simulink model "EV6_LUT_FourWheel_EV6Battery77p4kWh_PowerCorrected"  (R2024a)
settings: Solver=ode4  StartTime=0  StopTime=60  FixedStep=0.001  RelTol=1e-3
PreLoadFcn:
  | VSS_BICYCLE=Simulink.Variant('Dual=0');
  | VSS_DUAL=Simulink.Variant('Dual=1');
  | Dual=1;
  | load('DriveCycle2.mat')
PostLoadFcn:
  | if any(exist('dsrtsu_mdlpostloadfcn', 'file') ~= 0), dsrtsu_mdlpostloadfcn('Execute', bdroot); end
InitFcn:
  | , if any(exist('rtifpga_mdlclblib', 'file') ~= 0), rtifpga_mdlclblib('Init', bdroot); end,
  | , if any(exist('dsmpb_private', 'file') ~= 0), dsmpb_private('dsmpb_mdlclblib', 'Init', bdroot); end,
  | load('DriveCycle2.mat')
model workspace (MAT data in the model file):
  DiffRatio = 10.65
  EV6_2023_BattBranchCapacity_Ah = 55.5236728838
  EV6_2023_BattEnergy_kWh = 77.4
  EV6_2023_BattNominalVoltage_V = 697
  EV6_2023_BattNumCellsParallel = 2
  EV6_2023_BattNumCellsSeries = 192
  EV6_2023_BattOpenVoltCapBpts = [0 0.1 0.2 0.3 0.4 0.5 0.6 0.7 0.8 0.9 1]
  EV6_2023_BattOpenVoltTbl = [2.96762142548 3.40364281191 3.47417488548 3.54470541822 3.61523441014 3.68576186124 3.75628777151 3.82681214095 3.94527005036 4.07101207308 4.2120755254]
  EV6_2023_BattPackCapacity_Ah = 111.047345768
  EV6_2023_BattResistSocBpts = [0 0.2 0.4 0.6 0.8 1]
  EV6_2023_BattResistTbl = [0.0163620057716 0.0118174152018 0.00807187352333 0.00375663957972 0.00266904525531 0.00103635901355 0.0019014404175 0.0172368903217 0.0121226074867 0.00758541551769 0.00474065349228 0.00337561163613 ... (42 elements, 7x6)]
  EV6_2023_BattResistTempBpts = [243.1 253.1 263.1 273.1 283.1 298.1 313.1]
  EV6_2023_InitialPackOCV_V = 726.471714233
  EV6_2023_InitialSOC = 0.638878863672
  EV6_BattCellCapacity_Ah = 60.3
  EV6_BattInitialSOC = 0.638878863672
  EV6_BattOCV_Cell_V = [2.96762142548 3.40364281191 3.47417488548 3.54470541822 3.61523441014 3.68576186124 3.75628777151 3.82681214095 3.94527005036 4.07101207308 4.2120755254]
  EV6_BattOCV_SOC = [0 0.1 0.2 0.3 0.4 0.5 0.6 0.7 0.8 0.9 1]
  EV6_BattPackCapacity_Ah = 120.6
  EV6_BattParallelCells = 2
  EV6_BattResistanceSOC = [0 0.2 0.4 0.6 0.8 1]
  EV6_BattResistanceTable_Ohm = [0.0163620057716 0.0118174152018 0.00807187352333 0.00375663957972 0.00266904525531 0.00103635901355 0.0019014404175 0.0172368903217 0.0121226074867 0.00758541551769 0.00474065349228 0.00337561163613 ... (42 elements, 7x6)]
  EV6_BattResistanceTemp_K = [243.1 253.1 263.1 273.1 283.1 298.1 313.1]
  EV6_BattSeriesCells = 192
  EV6_FinalDriveRatio = 10.65
  EV6_TargetPackResistance_Ohm = 0.132763804608
  Gas = 0.383333333333
undefined symbols (not defined in the file): accel_bp_mps2, AccelCmd, ActTqLF_Nm_, ActTqLR_Nm_, ActTqRF_Nm_, ActTqRR_Nm_, BattChargeLimitMaxPwr, BattChargeLimitSocBpts, BattChargeLimitTbl, BattDischargeLimitSocBpts, BattDischargeLimitTbl, BattDischargeMaxPwr, BrakeMaxPrs, BrakeMaxTrq, ChassisDistCg2FrontAxle, ChassisDistCg2RearAxle, ChassisVehMass, CltchCmd, CoastDown, DecelCmd, DiscIntNeverNeededParam, EnvGravCnst, EnvPrs, EnvTemp, EV6_RegenTorqueGain, EV6_TractionTorqueGain, front_share_regen_3d, front_share_traction_3d, FuelSpecificGrav, GearCmd, h, InitStates, lgSw, limitedMCT, MCT, MtrEffSpdBpts, MtrEffTbl, MtrEffTrqBpts, MtrPwrMax, MtrTrqMax, out_1, pMCT, RealSimPara, Ref_speed, Ref_time, regen_torque_bp_Nm, speed_bp_kph, SteeringCmd, SupvsryCtrlRegenBrkCutOffTbl, SupvsryCtrlRegenSpdBpts, TestScnrioCycleNum, traction_torque_bp_Nm, US06, VEH
libraries: VSIGenLib x65, simulink x54, etargetslib x38, dsmpblib x24, vehdynlibtire x12, autolibshared x11, vehdynlibsuspension x7, vehdynlibtirecommon x7, autolibpowerinfoutils x6, autolibutils x5, autolibsharedcoupling x4, autolibmappedmotor x4
(part 11 of 19)

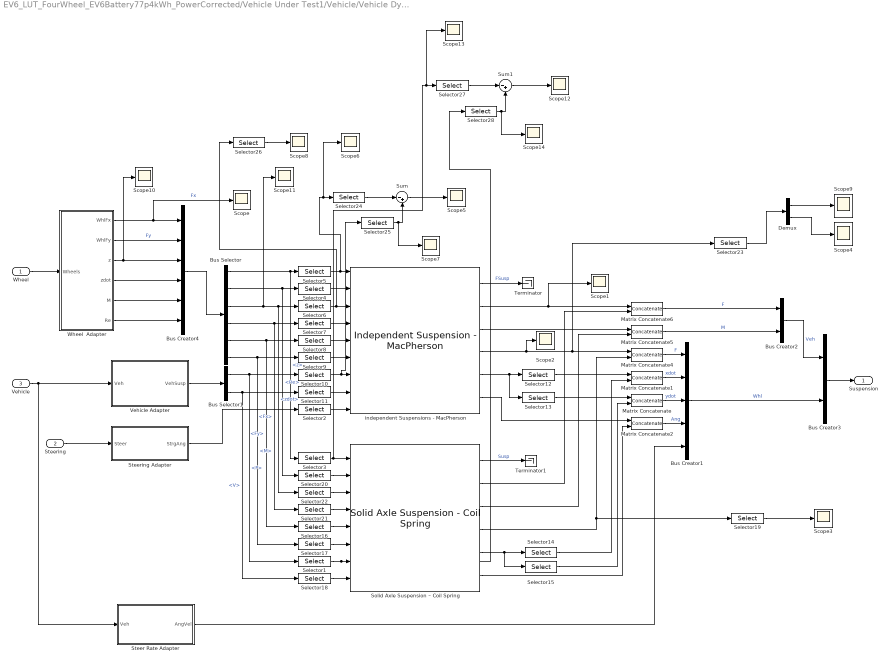
== system EV6_LUT_FourWheel_EV6Battery77p4kWh_PowerCorrected/Vehicle Under Test1/Vehicle/Vehicle Dynamics/Vehicle 14DOF/Suspension/MacPherson Front Suspension Solid Axle Rear Suspension ==
  Wheel : Inport
  Steering : Inport  Port=2
  Vehicle : Inport  Port=3
  Bus Creator1 : BusCreator  Inputs=5
  Bus Creator2 : BusCreator  Inputs=2
  Bus Creator3 : BusCreator  Inputs=2
  Bus Creator4 : BusCreator  Inputs=6
  Bus Selector : BusSelector  OutputSignals=z,Re,zdot,Fx,Fy,M
  Bus Selector1 : BusSelector  OutputSignals=P,V
  Demux : Demux  Outputs=2
  Matrix Concatenate{,1..2,4..6} (6 alike) : Concatenate  Mode=Multidimensional array  ConcatenateDimension=2
  Scope{,1..14} (15 alike) : Scope
  Selector1 : Selector  NumberOfDimensions=2  IndexOptions=Select all,Index vector (dialog)  Indices=[1 2],[3 4]  OutputSizes=1,1
  Selector10 : Selector  NumberOfDimensions=2  IndexOptions=Select all,Index vector (dialog)  Indices=[1 2],[1 2]  OutputSizes=1,1
  Selector11 : Selector  NumberOfDimensions=2  IndexOptions=Select all,Index vector (dialog)  Indices=[1 2],[1 2]  OutputSizes=1,1
  Selector12 : Selector  NumberOfDimensions=2  InputPortWidth=3  IndexOptions=Index vector (dialog),Select all  Indices=1,1  OutputSizes=1,1
  Selector13 : Selector  NumberOfDimensions=2  InputPortWidth=3  IndexOptions=Index vector (dialog),Select all  Indices=2,1  OutputSizes=1,1
  Selector14 : Selector  NumberOfDimensions=2  InputPortWidth=3  IndexOptions=Index vector (dialog),Select all  Indices=1,1  OutputSizes=1,1
  Selector15 : Selector  NumberOfDimensions=2  InputPortWidth=3  IndexOptions=Index vector (dialog),Select all  Indices=2,1  OutputSizes=1,1
  Selector{3,16,20..22} (5 alike) : Selector  IndexOptions=Index vector (dialog)  Indices=[3 4]  OutputSizes=1
  Selector17 : Selector  NumberOfDimensions=2  IndexOptions=Select all,Index vector (dialog)  Indices=[1 2],[3 4]  OutputSizes=1,1
  Selector18 : Selector  NumberOfDimensions=2  IndexOptions=Select all,Index vector (dialog)  Indices=[1 2],[3 4]  OutputSizes=1,1
  Selector19 : Selector  NumberOfDimensions=2  InputPortWidth=3  IndexOptions=Index vector (dialog),Select all  Indices=3,1  OutputSizes=1,1
  Selector{2,4..8} (6 alike) : Selector  IndexOptions=Index vector (dialog)  Indices=[1 2]  OutputSizes=1
  Selector23 : Selector  NumberOfDimensions=2  InputPortWidth=3  IndexOptions=Index vector (dialog),Select all  Indices=3,1  OutputSizes=1,1
  Selector24 : Selector  IndexOptions=Index vector (dialog)  Indices=[1]  OutputSizes=1
  Selector25 : Selector  NumberOfDimensions=2  IndexOptions=Index vector (dialog),Index vector (dialog)  Indices=[3],[1]  OutputSizes=1,1
  Selector26 : Selector  IndexOptions=Index vector (dialog)  Indices=[1]  OutputSizes=1
  Selector27 : Selector  IndexOptions=Index vector (dialog)  Indices=[1]  OutputSizes=1
  Selector28 : Selector  NumberOfDimensions=2  IndexOptions=Index vector (dialog),Index vector (dialog)  Indices=[3],[1]  OutputSizes=1,1
  Selector9 : Selector  NumberOfDimensions=2  IndexOptions=Select all,Index vector (dialog)  Indices=[1 2],[1 2]  OutputSizes=1,1
  Solid Axle Suspension – Coil Spring : vehdynlibsuspension/Solid Axle Suspension - Coil Spring  NumAxl=1  NumWhlsByAxl=2  StrgEnByAxl=0  WhlNumVec="[1  2]"  AxleNumVec="[1  1]"  SuspTypesByAxle=[1]  SuspImage=suspsacoil.png  AxlIxx=62  AxlM=160  TrackCoords=[0 0;1.9*[-1 1]/2;0 0]  SuspCoords=[0 0;1.9*[-1 1]/2;0 0]  KzWhlAxl=138031  F0zWhlAxl=5003*1  CzWhlAxl=11490  IdealSuspEn=on  IdealSuspAxles=[1]  Kz=52451*1  F0z=5003*1  Cz=5565*1  Hmax=0.32  Toe=0.  RollStrgSlp=0.  ToeStrgSlp=0  Caster=0.  CasterHslp=0.  CasterStrgSlp=0.01  Camber=0.  CamberHslp=0.  CamberStrgSlp=0.01  StrgHgtSlp=0.1432  MappedSuspEn=off  MappedSuspAxles="[1  2]"  f_susp_axl_bp=[1 2]  f_susp_dz_bp=[-0.15 -0.14 -0.13 -0.12 -0.11 -0.10 -0.09 -0.08 -0.07 -0.06 -0.05 -0.04 -0.03 -0.02 -0.01 0.00 0.01 0.02 0.03 0.04 0.05 0.06 0.07 0.08 0.09 0.10 0.11 0.12 0.13 0.14 0.15]  f_susp_dzdot_bp=[-0.15 -0.14 -0.13 -0.12 -0.11 -0.10 -0.09 -0.08 -0.07 -0.06 -0.05 -0.04 -0.03 -0.02 -0.01 0.00 0.01 0.02 0.03 0.04 0.05 0.06 0.07 0.08 0.09 0.10 0.11 0.12 0.13 0.14 0.15]  f_susp_fmz=zeros(31,31,61,2,4)  f_susp_geom=zeros(31,61,2,3)  f_susp_strgdelta_bp=[-30,-29,-28,-27,-26,-25,-24,-23,-22,-21,-20,-19,-18,-17,-16,-15,-14,-13,-12,-11,-10,-9,-8,-7,-6,-5,-4,-3,-2,-1,0,1,2,3,4,5,6,7,8,9,10,11,12,13,14,15,16,17,18,19,20,21,22,23,24,25,26,27,28,29,30]
  Steer Rate Adapter : Subsystem
  Steering Adapter : Subsystem
  Sum : Sum  Inputs=|-+
  Sum1 : Sum  Inputs=|-+
  Terminator : Terminator
  Terminator1 : Terminator
  Vehicle Adapter : Subsystem
  Wheel  Adapter : Subsystem
  independent Suspensions - MacPherson : vehdynlibsuspension/Independent Suspension - MacPherson  ActiveDampEn=off  NumAxl=1  NumWhlsByAxl=2  StrgEnByAxl=1  AntiSwayEnByAxl=1  WhlNumVec="[1  2]"  AxleNumVec="[1  1]"  SuspTypesByAxle=[1]  SuspImage=suspmacp.png  IdealSuspEn=on  IdealSuspAxles=[1]  Kz=52451*1  F0z=5003*1  Cz=5565*1  Hmax=0.32  f_act_susp_cz=[10000 10000;10000 10000]  f_act_susp_duty_bpt=[0 1]  f_act_susp_zdot_bpt=[-1 1]  Toe=0.  RollStrgSlp=0.  ToeStrgSlp=0.  Caster=0.  CasterHslp=0.  CasterStrgSlp=0.  Camber=0.  CamberHslp=0.  CamberStrgSlp=0.  StrgHgtSlp=0.1432  MappedSuspEn=off  MappedSuspAxles="[1  2]"  f_susp_axl_bp=[1 2]  f_susp_dz_bp=[-0.15 -0.14 -0.13 -0.12 -0.11 -0.10 -0.09 -0.08 -0.07 -0.06 -0.05 -0.04 -0.03 -0.02 -0.01 0.00 0.01 0.02 0.03 0.04 0.05 0.06 0.07 0.08 0.09 0.10 0.11 0.12 0.13 0.14 0.15]  f_susp_dzdot_bp=[-0.15 -0.14 -0.13 -0.12 -0.11 -0.10 -0.09 -0.08 -0.07 -0.06 -0.05 -0.04 -0.03 -0.02 -0.01 0.00 0.01 0.02 0.03 0.04 0.05 0.06 0.07 0.08 0.09 0.10 0.11 0.12 0.13 0.14 0.15]  f_susp_fmz=zeros(31,31,61,2,4)  f_susp_geom=zeros(31,61,2,3)  f_susp_strgdelta_bp=[-30,-29,-28,-27,-26,-25,-24,-23,-22,-21,-20,-19,-18,-17,-16,-15,-14,-13,-12,-11,-10,-9,-8,-7,-6,-5,-4,-3,-2,-1,0,1,2,3,4,5,6,7,8,9,10,11,12,13,14,15,16,17,18,19,20,21,22,23,24,25,26,27,28,29,30]  AntiSwayR=0.2  AntiSwayNtrlAng=0.5236  AntiSwayTrsK=8e+02
  Suspension : Outport  VectorParamsAs1DForOutWhenUnconnected=off
  wires:
  Steer Rate Adapter/1(AngVel) -> Bus Creator1/5
  Solid Axle Suspension – Coil Spring/5 -> Selector14/1, Selector15/1
  Solid Axle Suspension – Coil Spring/1 -> Terminator1/1  "Susp"
  Bus Selector/3 -> Scope11/1, Selector6/1, Selector22/1  "<zdot>"
  Selector22/1 -> Solid Axle Suspension – Coil Spring/3
  Vehicle/1 -> Vehicle Adapter/1(Veh), Steer Rate Adapter/1(Veh)
  Solid Axle Suspension – Coil Spring/3 -> Matrix Concatenate5/2
  Selector21/1 -> Solid Axle Suspension – Coil Spring/4
  Wheel  Adapter/6(Re) -> Bus Creator4/6
  Selector20/1 -> Solid Axle Suspension – Coil Spring/2
  Selector18/1 -> Solid Axle Suspension – Coil Spring/8
  Selector17/1 -> Solid Axle Suspension – Coil Spring/6
  Selector16/1 -> Solid Axle Suspension – Coil Spring/5
  Solid Axle Suspension – Coil Spring/2 -> Matrix Concatenate6/2
  Matrix Concatenate6/1 -> Bus Creator2/1  "F"
  Matrix Concatenate5/1 -> Bus Creator2/2  "M"
  Solid Axle Suspension – Coil Spring/4 -> Selector19/1, Matrix Concatenate4/2
  Matrix Concatenate4/1 -> Bus Creator1/1  "F"
  Solid Axle Suspension – Coil Spring/6 -> Matrix Concatenate2/2
  Matrix Concatenate2/1 -> Bus Creator1/4  "Ang"
  Selector14/1 -> Matrix Concatenate1/2
  Matrix Concatenate1/1 -> Bus Creator1/2  "xdot"
  Selector15/1 -> Matrix Concatenate/2
  Selector13/1 -> Matrix Concatenate/1
  Selector11/1 -> independent Suspensions - MacPherson/8
  Selector10/1 -> Selector25/1, independent Suspensions - MacPherson/7
  Selector9/1 -> independent Suspensions - MacPherson/6
  Selector8/1 -> independent Suspensions - MacPherson/5
  Selector7/1 -> independent Suspensions - MacPherson/4
  Selector6/1 -> Selector26/1, independent Suspensions - MacPherson/3
  Selector5/1 -> Scope6/1, Selector24/1, independent Suspensions - MacPherson/1
  Selector4/1 -> independent Suspensions - MacPherson/2
  Selector2/1 -> independent Suspensions - MacPherson/9
  Bus Selector/2 -> Selector4/1, Selector20/1  "<Re>"
  Wheel  Adapter/5(M) -> Bus Creator4/5
  Wheel  Adapter/4(zdot) -> Bus Creator4/4
  Wheel  Adapter/3(z) -> Scope10/1, Bus Creator4/3
  Wheel/1 -> Wheel  Adapter/1(Wheels)
  Wheel  Adapter/1(WhlFx) -> Bus Creator4/1, Scope/1  "Fx"
  Wheel  Adapter/2(WhlFy) -> Bus Creator4/2  "Fy"
  Bus Creator4/1 -> Bus Selector/1
  Steering Adapter/1(StrgAng) -> Selector2/1
  Bus Creator2/1 -> Bus Creator3/1  "Veh"
  independent Suspensions - MacPherson/3 -> Matrix Concatenate5/1
  independent Suspensions - MacPherson/2 -> Matrix Concatenate6/1, Scope1/1
  Vehicle Adapter/1(VehSusp) -> Bus Selector1/1
  Bus Selector/4 -> Selector21/1, Selector7/1  "<Fx>"
  independent Suspensions - MacPherson/1 -> Terminator/1  "FSusp"
  independent Suspensions - MacPherson/4 -> Selector23/1, Matrix Concatenate4/1, Scope2/1
  Selector12/1 -> Matrix Concatenate1/1
  independent Suspensions - MacPherson/6 -> Matrix Concatenate2/1
  independent Suspensions - MacPherson/5 -> Selector13/1, Selector12/1
  Matrix Concatenate/1 -> Bus Creator1/3  "ydot"
  Bus Selector1/1 -> Selector1/1, Selector10/1  "<P>"
  Steering/1 -> Steering Adapter/1(Steer)
  Bus Selector/1 -> Selector5/1, Selector3/1  "<z>"
  Bus Selector/5 -> Selector16/1, Selector8/1  "<Fy>"
  Bus Selector/6 -> Selector17/1, Selector9/1  "<M>"
  Bus Selector1/2 -> Selector18/1, Selector11/1  "<V>"
  Bus Creator1/1 -> Bus Creator3/2  "Whl"
  Bus Creator3/1 -> Suspension/1
  Selector19/1 -> Scope3/1
  Selector23/1 -> Demux/1
  Selector24/1 -> Sum/1
  Selector25/1 -> Scope7/1, Sum/2
  Sum/1 -> Scope5/1
  Selector26/1 -> Scope8/1
  Demux/1 -> Scope9/1
  Demux/2 -> Scope4/1
  Sum1/1 -> Scope12/1
  Selector28/1 -> Sum1/2, Scope14/1
  Selector27/1 -> Sum1/1
  Selector3/1 -> Solid Axle Suspension – Coil Spring/1, Selector27/1, Scope13/1
  Selector1/1 -> Solid Axle Suspension – Coil Spring/7, Selector28/1

== system EV6_LUT_FourWheel_EV6Battery77p4kWh_PowerCorrected/Vehicle Under Test1/Vehicle/Vehicle Dynamics/Vehicle 14DOF/Suspension/MacPherson Suspension ==
  Wheel : Inport
  Steering : Inport  Port=2
  Vehicle : Inport  Port=3
  Bus Creator1 : BusCreator  Inputs=5
  Bus Creator2 : BusCreator  Inputs=2
  Bus Creator3 : BusCreator  Inputs=2
  Bus Creator4 : BusCreator  Inputs=6
  Bus Selector : BusSelector  OutputSignals=z,Re,zdot,Fx,Fy,M
  Bus Selector1 : BusSelector  OutputSignals=P,V
  Selector1 : Selector  NumberOfDimensions=2  IndexOptions=Index vector (dialog),Select all  Indices=1,1  OutputSizes=1,1
  Selector2 : Selector  NumberOfDimensions=2  IndexOptions=Index vector (dialog),Select all  Indices=2,1  OutputSizes=1,1
  Steer Rate Adapter : Subsystem
  Steering Adapter : Subsystem
  Terminator : Terminator
  Vehicle Adapter : Subsystem
  Wheel  Adapter : Subsystem
  independent Suspensions - MacPherson : vehdynlibsuspension/Independent Suspension - MacPherson  ActiveDampEn=off  NumAxl=2  NumWhlsByAxl=[2 2]  StrgEnByAxl=[1 0]  AntiSwayEnByAxl=[1 0]  WhlNumVec="[1  2  1  2]"  AxleNumVec="[1  1  2  2]"  SuspTypesByAxle="[1  1]"  SuspImage=suspmacp.png  IdealSuspEn=on  IdealSuspAxles="[1  2]"  Kz=64370  F0z=9810  Cz=10000  Hmax=0.5  f_act_susp_cz=[10000 10000;10000 10000]  f_act_susp_duty_bpt=[0 1]  f_act_susp_zdot_bpt=[-1 1]  Toe=0.  RollStrgSlp=0.  ToeStrgSlp=0.  Caster=0.  CasterHslp=0.  CasterStrgSlp=0.  Camber=0.  CamberHslp=0.  CamberStrgSlp=0.  StrgHgtSlp=0.1432  MappedSuspEn=off  MappedSuspAxles="[1  2]"  f_susp_axl_bp=[1 2]  f_susp_dz_bp=[-0.15 -0.14 -0.13 -0.12 -0.11 -0.10 -0.09 -0.08 -0.07 -0.06 -0.05 -0.04 -0.03 -0.02 -0.01 0.00 0.01 0.02 0.03 0.04 0.05 0.06 0.07 0.08 0.09 0.10 0.11 0.12 0.13 0.14 0.15]  f_susp_dzdot_bp=[-0.15 -0.14 -0.13 -0.12 -0.11 -0.10 -0.09 -0.08 -0.07 -0.06 -0.05 -0.04 -0.03 -0.02 -0.01 0.00 0.01 0.02 0.03 0.04 0.05 0.06 0.07 0.08 0.09 0.10 0.11 0.12 0.13 0.14 0.15]  f_susp_fmz=zeros(31,31,61,2,4)  f_susp_geom=zeros(31,61,2,3)  f_susp_strgdelta_bp=[-30,-29,-28,-27,-26,-25,-24,-23,-22,-21,-20,-19,-18,-17,-16,-15,-14,-13,-12,-11,-10,-9,-8,-7,-6,-5,-4,-3,-2,-1,0,1,2,3,4,5,6,7,8,9,10,11,12,13,14,15,16,17,18,19,20,21,22,23,24,25,26,27,28,29,30]  AntiSwayR=0.2  AntiSwayNtrlAng=0.5236  AntiSwayTrsK=8e+02
  Suspension : Outport  VectorParamsAs1DForOutWhenUnconnected=off
  wires:
  independent Suspensions - MacPherson/1 -> Terminator/1  "Susp"
  Steering Adapter/1(StrgAng) -> independent Suspensions - MacPherson/9
  Steer Rate Adapter/1(AngVel) -> Bus Creator1/5  "AngVel"
  Bus Creator4/1 -> Bus Selector/1
  Bus Creator2/1 -> Bus Creator3/1  "Veh"
  independent Suspensions - MacPherson/2 -> Bus Creator2/1  "F"
  independent Suspensions - MacPherson/5 -> Selector1/1, Selector2/1  "V"
  independent Suspensions - MacPherson/6 -> Bus Creator1/4  "Ang"
  independent Suspensions - MacPherson/4 -> Bus Creator1/1  "F"
  Bus Selector/1 -> independent Suspensions - MacPherson/1  "<z>"
  Bus Selector1/1 -> independent Suspensions - MacPherson/7  "<P>"
  Selector2/1 -> Bus Creator1/3  "ydot"
  Selector1/1 -> Bus Creator1/2  "xdot"
  Bus Selector/2 -> independent Suspensions - MacPherson/2  "<Re>"
  Wheel  Adapter/6(Re) -> Bus Creator4/6
  Wheel  Adapter/5(M) -> Bus Creator4/5  "M"
  Wheel  Adapter/4(zdot) -> Bus Creator4/4
  Wheel  Adapter/3(z) -> Bus Creator4/3
  Wheel/1 -> Wheel  Adapter/1(Wheels)
  Wheel  Adapter/1(WhlFx) -> Bus Creator4/1  "Fx"
  Wheel  Adapter/2(WhlFy) -> Bus Creator4/2  "Fy"
  independent Suspensions - MacPherson/3 -> Bus Creator2/2  "M"
  Vehicle Adapter/1(VehSusp) -> Bus Selector1/1
  Vehicle/1 -> Vehicle Adapter/1(Veh), Steer Rate Adapter/1(Veh)
  Bus Selector/4 -> independent Suspensions - MacPherson/4  "<Fx>"
  Bus Selector/3 -> independent Suspensions - MacPherson/3  "<zdot>"
  Steering/1 -> Steering Adapter/1(Steer)
  Bus Selector/5 -> independent Suspensions - MacPherson/5  "<Fy>"
  Bus Selector/6 -> independent Suspensions - MacPherson/6  "<M>"
  Bus Selector1/2 -> independent Suspensions - MacPherson/8  "<V>"
  Bus Creator1/1 -> Bus Creator3/2  "Whl"
  Bus Creator3/1 -> Suspension/1

== system EV6_LUT_FourWheel_EV6Battery77p4kWh_PowerCorrected/Vehicle Under Test1/Vehicle/Vehicle Dynamics/Vehicle 14DOF/Suspension/Mapped Suspension ==
  Wheel : Inport
  Steering : Inport  Port=2
  Vehicle : Inport  Port=3
  Bus Creator1 : BusCreator  Inputs=5
  Bus Creator2 : BusCreator  Inputs=2
  Bus Creator3 : BusCreator  Inputs=2
  Bus Creator4 : BusCreator  Inputs=6
  Bus Selector : BusSelector  OutputSignals=z,Re,zdot,Fx,Fy,M
  Bus Selector1 : BusSelector  OutputSignals=P,V
  Independent Suspension - Mapped : vehdynlibsuspension/Independent Suspension - Mapped  NumAxl=2  NumWhlsByAxl=[2 2]  StrgEnByAxl=[1 0]  AntiSwayEnByAxl=[1 0]  WhlNumVec="[1  2  1  2]"  AxleNumVec="[1  1  2  2]"  SuspTypesByAxle="[2  2]"  SuspImage=suspindmap.png  IdealSuspEn=off  IdealSuspAxles="[1  2]"  Kz=64370  F0z=9810  Cz=10000  Hmax=0.5  Toe=2  RollStrgSlp=-13  ToeStrgSlp=0.01  Caster=4  CasterHslp=-13  CasterStrgSlp=0.01  Camber=4  CamberHslp=-13  CamberStrgSlp=0.01  StrgHgtSlp=0.0025  MappedSuspEn=on  MappedSuspAxles="[1  2]"  f_susp_axl_bp=[1 2]  f_susp_dz_bp=f_susp_dz_bp  f_susp_dzdot_bp=f_susp_dzdot_bp  f_susp_fmz=f_susp_fmz  f_susp_geom=f_susp_geom  f_susp_strgdelta_bp=f_susp_strgdelta_bp  NDFLookupOutType=1:4  NDGLookupOutType=1:3  AntiSwayR=0.2  AntiSwayNtrlAng=0.5236  AntiSwayTrsK=8e2
      link override For each track and axle combination calculate suspension forces and moments/Suspension/Suspension Angle Calculations: OverrideUsingVariant=MappedSteeringEnabled
      link override For each track and axle combination calculate suspension forces and moments/Suspension/Z axis suspension characteristic: OverrideUsingVariant=MappedSuspension
  Reshape1 : Reshape  OutputDimensionality=Row vector (2-D)
  Selector : Selector  IndexOptions=Index vector (dialog)  Indices=[1 2]  OutputSizes=1
  Selector1 : Selector  NumberOfDimensions=2  IndexOptions=Index vector (dialog),Select all  Indices=1,1  OutputSizes=1,1
  Selector2 : Selector  NumberOfDimensions=2  IndexOptions=Index vector (dialog),Select all  Indices=2,1  OutputSizes=1,1
  Steer Rate Adapter : Subsystem
  Terminator : Terminator
  Vehicle Adapter : Subsystem
  Wheel  Adapter : Subsystem
  Suspension : Outport  VectorParamsAs1DForOutWhenUnconnected=off
  wires:
  Steer Rate Adapter/1(AngVel) -> Bus Creator1/5
  Bus Creator3/1 -> Suspension/1
  Independent Suspension - Mapped/5 -> Selector1/1, Selector2/1  "V"
  Selector1/1 -> Bus Creator1/2  "xdot"
  Independent Suspension - Mapped/4 -> Bus Creator1/1  "F"
  Bus Creator1/1 -> Bus Creator3/2  "Whl"
  Bus Creator2/1 -> Bus Creator3/1  "Veh"
  Independent Suspension - Mapped/3 -> Bus Creator2/2  "M"
  Independent Suspension - Mapped/2 -> Bus Creator2/1  "F"
  Selector2/1 -> Bus Creator1/3  "ydot"
  Independent Suspension - Mapped/6 -> Bus Creator1/4  "Ang"
  Vehicle/1 -> Vehicle Adapter/1(Veh), Steer Rate Adapter/1(Veh)
  Steering/1 -> Selector/1
  Bus Selector1/1 -> Independent Suspension - Mapped/7  "<P>"
  Wheel  Adapter/1(WhlFx) -> Bus Creator4/1  "Fx"
  Bus Selector/1 -> Independent Suspension - Mapped/1  "<z>"
  Bus Selector/3 -> Independent Suspension - Mapped/3  "<zdot>"
  Vehicle Adapter/1(VehSusp) -> Bus Selector1/1
  Wheel/1 -> Wheel  Adapter/1(Wheels)
  Wheel  Adapter/2(WhlFy) -> Bus Creator4/2  "Fy"
  Wheel  Adapter/3(z) -> Bus Creator4/3
  Bus Creator4/1 -> Bus Selector/1
  Selector/1 -> Reshape1/1
  Wheel  Adapter/6(Re) -> Bus Creator4/6
  Wheel  Adapter/4(zdot) -> Bus Creator4/4
  Bus Selector/6 -> Independent Suspension - Mapped/6  "<M>"
  Wheel  Adapter/5(M) -> Bus Creator4/5
  Bus Selector/4 -> Independent Suspension - Mapped/4  "<Fx>"
  Bus Selector1/2 -> Independent Suspension - Mapped/8  "<V>"
  Bus Selector/2 -> Independent Suspension - Mapped/2  "<Re>"
  Bus Selector/5 -> Independent Suspension - Mapped/5  "<Fy>"
  Reshape1/1 -> Independent Suspension - Mapped/9
  Independent Suspension - Mapped/1 -> Terminator/1  "Susp"

== system EV6_LUT_FourWheel_EV6Battery77p4kWh_PowerCorrected/Vehicle Under Test1/Vehicle/Vehicle Dynamics/Vehicle 14DOF/Vehicle/Variant Subsystem ==
  note: 1) Add Subsystem or Model blocks as valid variant choices.
      | 2) You cannot connect blocks at this level. At simulation, connectivity is automatically
      | determined, based on the active variant and port name matching.
  Suspension : Inport
  Wind : Inport  Port=2
  3DOF : Subsystem  VariantControl=0
  6DOF : Subsystem  VariantControl=1
  VehFdbk : Outport  VectorParamsAs1DForOutWhenUnconnected=off

== system EV6_LUT_FourWheel_EV6Battery77p4kWh_PowerCorrected/Vehicle Under Test1/Vehicle/Vehicle Dynamics/Vehicle 14DOF/Wheels and Tires/VDBS ==
  WheelAng : Inport
  CamberAng : Inport  Port=2  Unit=rad
  AxleTrq : Inport  Port=3
  BrkPrs : Inport  Port=4
  Fz : Inport  Port=5  Unit=N
  r : Inport  Port=6
  VehVel : Inport  Port=7
  Ground Level : Inport  Port=8
  Friction : Inport  Port=9  Unit=1  PortDimensions=4
  Bus Selector : BusSelector  OutputSignals=z
  Pressure : vehdynlibtirecommon/Constant  const=220000  numWheels=4
  Scope{,1..4} (5 alike) : Scope
  Terminator : Terminator
  Tire2Veh : Subsystem
  Tires : Subsystem  Variant=on  VariantControlMode=label  VariantControl=Variant1  LabelModeActiveChoice=0
  Veh2Tire : Subsystem
  scale factors with friction : Subsystem  mask{numWheels=4}
      mask prompts: numWheels "Number of wheels"
  Wheels : Outport  VectorParamsAs1DForOutWhenUnconnected=off
  FrntAxlF : Outport  Port=2  Unit=N  VectorParamsAs1DForOutWhenUnconnected=off
  RearAxlF : Outport  Port=3  Unit=N  VectorParamsAs1DForOutWhenUnconnected=off
  Omega : Outport  Port=4  VectorParamsAs1DForOutWhenUnconnected=off
  Mz : Outport  Port=5  Unit=N*m  VectorParamsAs1DForOutWhenUnconnected=off
  SuspWhlPz : Outport  Port=6  VectorParamsAs1DForOutWhenUnconnected=off
  SuspWhlVz : Outport  Port=7  VectorParamsAs1DForOutWhenUnconnected=off
  wires:
  Tire2Veh/1(Wheels) -> Wheels/1
  CamberAng/1 -> Veh2Tire/6(WheelCamber), Tire2Veh/3(WheelCamber), Tires/6("Camber ")
  Tire2Veh/7(SuspWhlVz) -> SuspWhlVz/1
  Tire2Veh/6(SuspWhlPz) -> SuspWhlPz/1
  Veh2Tire/6(zdotAxle) -> Terminator/1
  r/1 -> Veh2Tire/1(r)
  Friction/1 -> scale factors with friction/2(lamda_mu_y), scale factors with friction/1(lamda_mu_x)
  Tire2Veh/5(<Mz>) -> Mz/1
  Tire2Veh/4(RearAxlF) -> RearAxlF/1
  Tire2Veh/3(FrntAxlF) -> FrntAxlF/1
  Tire2Veh/2(Omega) -> Omega/1, Scope/1
  WheelAng/1 -> Tire2Veh/4(WheelSteer), Veh2Tire/5(WheelSteer)
  Tires/1(" Wheels") -> Bus Selector/1, Tire2Veh/1(Wheel)
  Veh2Tire/3(psidot) -> Tires/3("r ")
  Veh2Tire/5(ydotAxle) -> Tires/5("Vy ")
  Veh2Tire/4(xdotAxle) -> Tires/4("Vx ")
  Veh2Tire/2(P) -> Tires/2("Brake Pressure ")
  Veh2Tire/1(T) -> Scope1/1, Tires/1("DriveTorque ")
  VehVel/1 -> Veh2Tire/4(VehVel)
  BrkPrs/1 -> Veh2Tire/3(Brake)
  AxleTrq/1 -> Scope2/1, Veh2Tire/2(Axle)
  Fz/1 -> Tire2Veh/2(Fz), Tires/10("FzSusp ")
  scale factors with friction/1(lambdas) -> Tires/8("lambda ")
  Pressure/1 -> Tires/7("Press ")
  Ground Level/1 -> Scope3/1, Tires/9("Gnd ")
  Bus Selector/1 -> Scope4/1  "<z>"

== system EV6_LUT_FourWheel_EV6Battery77p4kWh_PowerCorrected/Vehicle Under Test1/Vehicle/Vehicle Dynamics/Vehicle 7DOF/Longitudinal Wheels 4DOF/Axle Forces ==
  note: 1) Add Subsystem or Model blocks as valid variant choices.
      | 2) You cannot connect blocks at this level. At simulation, connectivity is automatically
      | determined, based on the active variant and port name matching.
  F : Inport
  R : Inport  Port=2
  Bicycle : Subsystem  VariantControl=0
  Dual : Subsystem  VariantControl=1
  FrntAxlF : Outport  Unit=N  VectorParamsAs1DForOutWhenUnconnected=off
  RearAxlF : Outport  Port=2  Unit=N  VectorParamsAs1DForOutWhenUnconnected=off

== system EV6_LUT_FourWheel_EV6Battery77p4kWh_PowerCorrected/Vehicle Under Test1/Vehicle/Vehicle Dynamics/Vehicle 7DOF/Longitudinal Wheels 4DOF/Tire2Veh ==
  Wheel : Inport
  Bus Selector7 : BusSelector  OutputSignals=Omega,Fx,Re,z,zdot,Kappa,Alpha
  Dead Zone2 : DeadZone  LowerValue=-5  UpperValue=5  ZeroCross=off
  Demux : Demux  Outputs=[2,2]
  Re : Terminator
  Unary Minus1 : UnaryMinus
  Unary Minus2 : UnaryMinus
  zdot : Terminator
  FwF : Outport  VectorParamsAs1DForOutWhenUnconnected=off
  FwR : Outport  Port=2  VectorParamsAs1DForOutWhenUnconnected=off
  z : Outport  Port=3  VectorParamsAs1DForOutWhenUnconnected=off
  Omega : Outport  Port=4  VectorParamsAs1DForOutWhenUnconnected=off
  Kappa : Outport  Port=5  VectorParamsAs1DForOutWhenUnconnected=off
  Alpha : Outport  Port=6  VectorParamsAs1DForOutWhenUnconnected=off
  wires:
  Bus Selector7/7 -> Alpha/1  "<Alpha>"
  Bus Selector7/3 -> Re/1  "<Re>"
  Unary Minus2/1 -> zdot/1  "zdot"
  Bus Selector7/6 -> Kappa/1  "<Kappa>"
  Demux/2 -> FwR/1
  Unary Minus1/1 -> z/1  "z"
  Bus Selector7/4 -> Unary Minus1/1  "<z>"
  Bus Selector7/5 -> Unary Minus2/1  "<zdot>"
  Bus Selector7/1 -> Omega/1  "<Omega>"
  Wheel/1 -> Bus Selector7/1
  Demux/1 -> FwF/1
  Dead Zone2/1 -> Demux/1  "Fx"
  Bus Selector7/2 -> Dead Zone2/1  "<Fx>"

== system EV6_LUT_FourWheel_EV6Battery77p4kWh_PowerCorrected/Vehicle Under Test1/Vehicle/Vehicle Dynamics/Vehicle 7DOF/Longitudinal Wheels 4DOF/Tires ==
  AxlTrq : Inport
  BrkPrs : Inport  Port=2
  Vx : Inport  Port=3
  Vy : Inport  Port=4
  r : Inport  Port=5
  Camber : Inport  Port=6
  TirePrs : Inport  Port=7
  Fz : Inport  Port=8
  lam_mu : Inport  Port=9
  Gnd : Inport  Port=10
  4-by-1 Gnd : Subsystem
  4-by-1 Gnd1 : Subsystem
  4-by-1 Gnd2 : Subsystem
  4-by-1 Gnd3 : Subsystem
  Bus Creator : BusCreator  Inputs=12
  Subsystem : Subsystem
  Terminator1 : Terminator
  Terminator2 : Terminator
  Terminator3 : Terminator
  Wheel : Outport  VectorParamsAs1DForOutWhenUnconnected=off
  wires:
  Gnd/1 -> Subsystem/7(Gnd)
  lam_mu/1 -> Subsystem/6(lam_mu)
  Fz/1 -> Subsystem/5(Fz)
  TirePrs/1 -> Subsystem/4(TirePrs)
  Vx/1 -> Subsystem/3(Vx)
  BrkPrs/1 -> Subsystem/2(BrkPrs)
  AxlTrq/1 -> Subsystem/1(AxlTrq)
  4-by-1 Gnd3/1(Gnd) -> Bus Creator/12  "Alpha"
  Subsystem/8(Kappa) -> Bus Creator/11  "Kappa"
  4-by-1 Gnd2/1(Gnd) -> Bus Creator/7  "Mz"
  4-by-1 Gnd1/1(Gnd) -> Bus Creator/5  "Mx"
  4-by-1 Gnd/1(Gnd) -> Bus Creator/3  "Fy"
  Subsystem/4(My) -> Bus Creator/6  "My"
  Subsystem/3(FzOut) -> Bus Creator/4  "Fz"
  Subsystem/5(Re) -> Bus Creator/8  "Re"
  Subsystem/1(Omega) -> Bus Creator/1  "Omega"
  Subsystem/2(Fx) -> Bus Creator/2  "Fx"
  Subsystem/6(z) -> Bus Creator/9  "z"
  Subsystem/7(zdot) -> Bus Creator/10  "zdot"
  Bus Creator/1 -> Wheel/1
  r/1 -> Terminator3/1
  Camber/1 -> Terminator2/1
  Vy/1 -> Terminator1/1

== system EV6_LUT_FourWheel_EV6Battery77p4kWh_PowerCorrected/Vehicle Under Test1/Vehicle/Vehicle Dynamics/Vehicle 7DOF/Longitudinal Wheels 4DOF/Veh2Tire ==
  AxlTrq : Inport
  BrkPrs : Inport  Port=2
  r : Inport  Port=3
  VehVel : Inport  Port=4
  WhlAng : Inport  Port=5
  Reshape3 : Reshape
  Reshape4 : Reshape
  Unary Minus : UnaryMinus
  Wheel to Body Transform : Subsystem
  T : Outport  VectorParamsAs1DForOutWhenUnconnected=off
  P : Outport  Port=2  VectorParamsAs1DForOutWhenUnconnected=off
  xdotAxle : Outport  Port=3  VectorParamsAs1DForOutWhenUnconnected=off
  ydotAxle : Outport  Port=4  VectorParamsAs1DForOutWhenUnconnected=off
  psidot : Outport  Port=5  VectorParamsAs1DForOutWhenUnconnected=off
  zdotAxle : Outport  Port=6  VectorParamsAs1DForOutWhenUnconnected=off
  wires:
  Reshape3/1 -> P/1
  Unary Minus/1 -> psidot/1
  Wheel to Body Transform/3(zdotWheel) -> zdotAxle/1  "Vz"
  WhlAng/1 -> Wheel to Body Transform/2(WhlAng)
  VehVel/1 -> Wheel to Body Transform/1(VelVeh)
  Reshape4/1 -> T/1
  r/1 -> Unary Minus/1
  Wheel to Body Transform/2(ydotWheel) -> ydotAxle/1  "Vy"
  Wheel to Body Transform/1(xdotWheel) -> xdotAxle/1  "Vx"
  AxlTrq/1 -> Reshape4/1
  BrkPrs/1 -> Reshape3/1

== system EV6_LUT_FourWheel_EV6Battery77p4kWh_PowerCorrected/Vehicle Under Test1/Vehicle/Vehicle Dynamics/Vehicle 7DOF/Longitudinal Wheels 4DOF/Velocity and Vertical Load ==
  note: 1) Add Subsystem or Model blocks as valid variant choices.
      | 2) You cannot connect blocks at this level. At simulation, connectivity is automatically
      | determined, based on the active variant and port name matching.
  VehFdbk : Inport
  Bicycle : Subsystem  VariantControl=0
  Dual : Subsystem  VariantControl=1
  VehVel : Outport  VectorParamsAs1DForOutWhenUnconnected=off
  Fz : Outport  Port=2  PortDimensions=4  VectorParamsAs1DForOutWhenUnconnected=off

== system EV6_LUT_FourWheel_EV6Battery77p4kWh_PowerCorrected/Vehicle Under Test1/Vehicle/Vehicle Dynamics/Vehicle 7DOF/Longitudinal Wheels 4DOF/Wheel Angles ==
  WheelAng : Inport
  Camber : Inport  Port=2
  Add1 : Sum
  Constant2 : Constant  Value=0
  Constant3 : Constant  Value=ones(1,4).*pi
  Demux : Demux  Outputs=2
  Demux1 : Demux
  Mux : Mux  Inputs=2
  Reshape : Reshape  OutputDimensionality=Row vector (2-D)
  Reshape1 : Reshape  OutputDimensionality=Row vector (2-D)
  Reshape2 : Reshape  OutputDimensionality=Row vector (2-D)
  Vector Concatenate3 : Concatenate  NumInputs=3  Mode=Multidimensional array
  Vector Concatenate4 : Concatenate  NumInputs=4
  WhlAngB : Outport  VectorParamsAs1DForOutWhenUnconnected=off
  wires:
  WheelAng/1 -> Demux1/1
  Camber/1 -> Reshape2/1
  Reshape2/1 -> Vector Concatenate3/2
  Reshape1/1 -> Vector Concatenate3/1
  Reshape/1 -> Vector Concatenate3/3
  Vector Concatenate3/1 -> WhlAngB/1
  Constant3/1 -> Reshape1/1
  Vector Concatenate4/1 -> Reshape/1
  Demux/2 -> Vector Concatenate4/4
  Demux/1 -> Vector Concatenate4/2
  Demux1/4 -> Mux/2
  Mux/1 -> Add1/1
  Demux1/1 -> Vector Concatenate4/1
  Demux1/3 -> Vector Concatenate4/3
  Add1/1 -> Demux/1
  Constant2/1 -> Add1/2
  Demux1/2 -> Mux/1

== system EV6_LUT_FourWheel_EV6Battery77p4kWh_PowerCorrected/Vehicle Under Test1/Vehicle/Vehicle Dynamics/Vehicle 7DOF/Subsystem4/Subsystem ==
  CgXYZdot : Inport
  angles : Inport  Port=2
  Demux2 : Demux  Outputs=3
  Demux3 : Demux  Outputs=3
  Terminator{,1..4} (5 alike) : Terminator
  VehSpd : Outport
  wires:
  Demux2/1 -> VehSpd/1  "Xdot"
  angles/1 -> Demux3/1
  Demux2/3 -> Terminator1/1  "Zdot"
  Demux3/3 -> Terminator4/1  "psi"
  Demux3/1 -> Terminator2/1  "phi"
  Demux2/2 -> Terminator/1  "Ydot"
  Demux3/2 -> Terminator3/1  "theta"
  CgXYZdot/1 -> Demux2/1

== system EV6_LUT_FourWheel_EV6Battery77p4kWh_PowerCorrected/Vehicle Under Test1/Vehicle/Vehicle Dynamics/Vehicle 7DOF/Vehicle Body 3DOF External Longitudinal Wheels/Bicycle ==
  WhlAng : Inport
  "FwF " : Inport  Port=2
  "FwR " : Inport  Port=3
  WindXYZ : Inport  Port=4
  Friction : Inport  Port=5
  Demux : Demux  Outputs=[2,2]
  Gain : Gain  Gain=.5
  Gain1 : Gain  Gain=.5
  Gain2 : Gain  Gain=.5
  Selector : Selector  InputPortWidth=4  IndexOptions=Index vector (dialog)  Indices=[1 2]  OutputSizes=1
  Signal Specification : SignalSpecification  Unit=1
  Signal Specification1 : SignalSpecification  Unit=rad
  Sum of Elements : Sum  Inputs=+
  Sum of Elements1 : Sum  Inputs=+
  Sum of Elements2 : Sum  Inputs=+
  Terminator{,1..5} (6 alike) : Terminator
  Vector Concatenate : Concatenate
  Vehicle Body 3DOF Single Track : autolibshared/Vehicle Body 3DOF Single Track  trackMode=Single (bicycle)  inputMode=External longitudinal forces  frontSteerMode=on  rearSteerMode=off  windMode=on  muMode=on  extFMode=off  extMMode=off  htchFMode=off  htchMMode=off  extXo=off  extpsio=off  extxdoto=off  extro=off  extYo=off  extTamb=off  extydoto=off  aMode=2  NF=ChassisNumFrontWhls  NR=ChassisNumRearWhls  m=ChassisVehMass  a=ChassisDistCg2FrontAxle  b=ChassisDistCg2RearAxle  h=ChassisCgHeight  dh=1  hh=0.2  X_o=0  xdot_o=20  CalphaMode=off  sigmaMode=on  d=0  hl=0  w=1.922.*[1 1]  Cy_f=15000  Cy_r=35000  sigma_f=.1  sigma_r=.1  alpha_f_brk=[-.1 .1]  Cy_f_data=[-9e3 9e3]  alpha_r_brk=[-.1 .1]  Cy_r_data=[-9e3 9e3]  Y_o=0  ydot_o=0  Izz=2500  psi_o=0  r_o=0  Af=ChassisFrontalArea  Cd=ChassisDragCoeff  Cl=.1  Cpm=.1  beta_w=[0:0.01:0.3]  Cs=[0:0.03:0.9]  Cym=[0:0.01:0.3]  Pabs=EnvPrs  Tair=EnvTemp  g=EnvGravCnst  mu=1  xdot_tol=1  Fznom=5000  Fxtire_sat=7e3*1e3  Fytire_sat=2e3*1e3  longOff=0  latOff=0  vertOff=.0112  wrapAng=off
  Wheel Positions : Subsystem
  " Info" : Outport  VectorParamsAs1DForOutWhenUnconnected=off
  XWheel : Outport  Port=2  Unit=m  VectorParamsAs1DForOutWhenUnconnected=off
  " YWheel" : Outport  Port=3  Unit=m  VectorParamsAs1DForOutWhenUnconnected=off
  wires:
  Vehicle Body 3DOF Single Track/3 -> Terminator5/1
  Vehicle Body 3DOF Single Track/2 -> Terminator4/1
  Vehicle Body 3DOF Single Track/5 -> Terminator3/1
  Vehicle Body 3DOF Single Track/4 -> Terminator2/1
  Wheel Positions/1(XWheel) -> XWheel/1
  Wheel Positions/2(YWheel) -> " YWheel"/1
  Signal Specification1/1 -> Vehicle Body 3DOF Single Track/1
  Signal Specification/1 -> ?
  Vector Concatenate/1 -> Signal Specification/1
  Gain2/1 -> Vector Concatenate/2
  Gain1/1 -> Vector Concatenate/1
  Demux/2 -> Sum of Elements2/1
  Sum of Elements2/1 -> Gain2/1
  Sum of Elements1/1 -> Gain1/1
  Friction/1 -> Demux/1
  Demux/1 -> Sum of Elements1/1
  Selector/1 -> Sum of Elements/1
  WindXYZ/1 -> ?
  Vehicle Body 3DOF Single Track/7 -> Terminator1/1
  Vehicle Body 3DOF Single Track/6 -> Terminator/1
  Sum of Elements/1 -> Gain/1
  Gain/1 -> Signal Specification1/1
  WhlAng/1 -> Selector/1
  Vehicle Body 3DOF Single Track/1 -> Wheel Positions/1(Info), " Info"/1
  "FwF "/1 -> Vehicle Body 3DOF Single Track/2
  "FwR "/1 -> Vehicle Body 3DOF Single Track/3

== system EV6_LUT_FourWheel_EV6Battery77p4kWh_PowerCorrected/Vehicle Under Test1/Vehicle/Vehicle Dynamics/Vehicle 7DOF/Vehicle Body 3DOF External Longitudinal Wheels/Dual ==
  WhlAng : Inport
  "FwF " : Inport  Port=2
  "FwR " : Inport  Port=3
  WindXYZ : Inport  Port=4
  Friction : Inport  Port=5
  Reshape : Reshape  OutputDimensionality=Customize  OutputDimensions=[2,2]
  Selector : Selector  InputPortWidth=4  IndexOptions=Index vector (dialog)  Indices=[1 2]  OutputSizes=1
  Signal Specification : SignalSpecification  Unit=1
  Terminator{,1..5} (6 alike) : Terminator
  Vehicle Body 3DOF Dual Track : autolibshared/Vehicle Body 3DOF Single Track  trackMode=Dual  inputMode=External longitudinal forces  frontSteerMode=on  rearSteerMode=off  windMode=on  muMode=on  extFMode=off  extMMode=off  htchFMode=off  htchMMode=off  extXo=off  extpsio=off  extxdoto=off  extro=off  extYo=off  extTamb=off  extydoto=off  aMode=2  NF=ChassisNumFrontWhls  NR=ChassisNumRearWhls  m=ChassisVehMass  a=ChassisDistCg2FrontAxle  b=ChassisDistCg2RearAxle  h=ChassisCgHeight  dh=1  hh=0.2  X_o=0  xdot_o=InitStates(TestScnrioCycleNum).VehSpd  CalphaMode=off  sigmaMode=on  d=0  hl=0  w=1.9.*[1 1]  Cy_f=15000  Cy_r=35000  sigma_f=.1  sigma_r=.1  alpha_f_brk=[-.1 .1]  Cy_f_data=[-9e3 9e3]  alpha_r_brk=[-.1 .1]  Cy_r_data=[-9e3 9e3]  Y_o=0  ydot_o=0  Izz=2500  psi_o=0  r_o=0  Af=ChassisFrontalArea  Cd=ChassisDragCoeff  Cl=.1  Cpm=.1  beta_w=[0:0.01:0.3]  Cs=[0:0.03:0.9]  Cym=[0:0.01:0.3]  Pabs=EnvPrs  Tair=EnvTemp  g=EnvGravCnst  mu=1  xdot_tol=1  Fznom=5000  Fxtire_sat=7e3*1e3  Fytire_sat=2e3*1e3  longOff=0  latOff=0  vertOff=.0112  wrapAng=off
  Wheel Positions : Subsystem
  " Info" : Outport  VectorParamsAs1DForOutWhenUnconnected=off
  " XWheel" : Outport  Port=2  VectorParamsAs1DForOutWhenUnconnected=off
  " YWheel" : Outport  Port=3  VectorParamsAs1DForOutWhenUnconnected=off
  wires:
  "FwR "/1 -> Vehicle Body 3DOF Dual Track/3
  "FwF "/1 -> Vehicle Body 3DOF Dual Track/2
  WindXYZ/1 -> ?
  Signal Specification/1 -> ?
  Vehicle Body 3DOF Dual Track/7 -> Terminator/1
  Vehicle Body 3DOF Dual Track/5 -> Terminator3/1
  Vehicle Body 3DOF Dual Track/4 -> Terminator2/1
  Vehicle Body 3DOF Dual Track/6 -> Terminator1/1
  Vehicle Body 3DOF Dual Track/3 -> Terminator5/1
  Vehicle Body 3DOF Dual Track/2 -> Terminator4/1
  Wheel Positions/2(YWheel) -> " YWheel"/1
  Wheel Positions/1(XWheel) -> " XWheel"/1
  Vehicle Body 3DOF Dual Track/1 -> Wheel Positions/1(Info), " Info"/1
  Reshape/1 -> Signal Specification/1
  Friction/1 -> Reshape/1
  Selector/1 -> Vehicle Body 3DOF Dual Track/1
  WhlAng/1 -> Selector/1

== system EV6_LUT_FourWheel_EV6Battery77p4kWh_PowerCorrected/Vehicle Under Test1/Vehicle/Vehicle Dynamics/Vehicle Longitudinal/Longitudinal Wheels/Front Diff Wheels ==
  BrkPrs : Inport
  AxleTorq : Inport  Port=2
  Add2 : Sum
  Bus Creator : BusCreator  Inputs=3
  Bus Creator5 : BusCreator  Inputs=1
  Bus Selector6 : BusSelector  OutputSignals=VehSpd,FrcZ
  Bus Selector7 : BusSelector  OutputSignals=VehSpd,FrcZ
  Selector : Selector  InputPortWidth=4  IndexOptions=Index vector (dialog)  Indices=1  OutputSizes=1
  Selector1 : Selector  InputPortWidth=4  IndexOptions=Index vector (dialog)  Indices=2  OutputSizes=1
  Selector2 : Selector  InputPortWidth=4  IndexOptions=Index vector (dialog)  Indices=1  OutputSizes=1
  Selector3 : Selector  InputPortWidth=4  IndexOptions=Index vector (dialog)  Indices=2  OutputSizes=1
  Simple Longitudinal Wheel 1 : VsrLibWheel/Simple Longitudinal Wheel  TireLoadedRadius=WhlRearLoadedRadius  C_rr=WhlRollingResistCnst  MaxBrkTrq=BrakeMaxTrq  MaxBrkPrs=BrakeMaxPrs  w_thresh=WhlSimVelTol
  Simple Longitudinal Wheel 2 : VsrLibWheel/Simple Longitudinal Wheel  TireLoadedRadius=WhlRearLoadedRadius  C_rr=WhlRollingResistCnst  MaxBrkTrq=BrakeMaxTrq  MaxBrkPrs=BrakeMaxPrs  w_thresh=WhlSimVelTol
  Terminator3 : Terminator
  Two-Way Connection6 : TwoWayConnection
  DiffAxle : PMIOPort  Side=Right
  Info : Outport
  wires:
  Simple Longitudinal Wheel 2/3 -> Bus Creator/3  "Omega2"
  Simple Longitudinal Wheel 1/1 -> Bus Creator/1  "WhlFrontInfo"
  Bus Creator/1 -> Info/1
  Simple Longitudinal Wheel 1/3 -> Bus Creator/2  "Omega1"
  Selector3/1 -> Simple Longitudinal Wheel 2/1
  Selector1/1 -> Simple Longitudinal Wheel 2/2
  Selector/1 -> Simple Longitudinal Wheel 1/2
  AxleTorq/1 -> Selector/1, Selector1/1
  Selector2/1 -> Simple Longitudinal Wheel 1/1
  Simple Longitudinal Wheel 2/1 -> Terminator3/1
  Bus Creator5/1 -> Two-Way Connection6/1
  Simple Longitudinal Wheel 2/2 -> Add2/2  "Spd"
  Add2/1 -> Bus Creator5/1  "FrcX"
  Two-Way Connection6/1 -> Bus Selector6/1, Bus Selector7/1
  Bus Selector7/2 -> Simple Longitudinal Wheel 2/4  "<FrcZ>"
  Bus Selector6/1 -> Simple Longitudinal Wheel 1/3  "<VehSpd>"
  Bus Selector7/1 -> Simple Longitudinal Wheel 2/3  "<VehSpd>"
  Simple Longitudinal Wheel 1/2 -> Add2/1
  BrkPrs/1 -> Selector2/1, Selector3/1
  Bus Selector6/2 -> Simple Longitudinal Wheel 1/4  "<FrcZ>"
  connections:
  DiffAxle/RConn1 -- Two-Way Connection6/RConn1

== system EV6_LUT_FourWheel_EV6Battery77p4kWh_PowerCorrected/Vehicle Under Test1/Vehicle/Vehicle Dynamics/Vehicle Longitudinal/Longitudinal Wheels/Rear Wheels ==
  BrkPrs : Inport
  Add2 : Sum
  Bus Creator : BusCreator  Inputs=3
  Bus Creator5 : BusCreator  Inputs=1
  Bus Selector6 : BusSelector  OutputSignals=VehSpd,FrcZ
  Bus Selector7 : BusSelector  OutputSignals=VehSpd,FrcZ
  Ground : Ground
  Selector : Selector  InputPortWidth=4  IndexOptions=Index vector (dialog)  Indices=3  OutputSizes=1
  Selector1 : Selector  InputPortWidth=4  IndexOptions=Index vector (dialog)  Indices=4  OutputSizes=1
  Simple Longitudinal Wheel : VsrLibWheel/Simple Longitudinal Wheel  TireLoadedRadius=WhlFrontLoadedRadius  C_rr=WhlRollingResistCnst  MaxBrkTrq=BrakeMaxTrq  MaxBrkPrs=BrakeMaxPrs  w_thresh=WhlSimVelTol
  Simple Longitudinal Wheel1 : VsrLibWheel/Simple Longitudinal Wheel  TireLoadedRadius=WhlFrontLoadedRadius  C_rr=WhlRollingResistCnst  MaxBrkTrq=BrakeMaxTrq  MaxBrkPrs=BrakeMaxPrs  w_thresh=WhlSimVelTol
  Terminator3 : Terminator
  Two-Way Connection6 : TwoWayConnection
  DiffAxle : PMIOPort  Side=Right
  Info : Outport
  wires:
  Bus Creator/1 -> Info/1
  Simple Longitudinal Wheel/1 -> Bus Creator/1  "WhlRearInfo"
  Selector1/1 -> Simple Longitudinal Wheel1/1
  Selector/1 -> Simple Longitudinal Wheel/1
  Bus Selector6/2 -> Simple Longitudinal Wheel/4  "<FrcZ>"
  BrkPrs/1 -> Selector/1, Selector1/1
  Simple Longitudinal Wheel/2 -> Add2/1
  Bus Selector7/1 -> Simple Longitudinal Wheel1/3  "<VehSpd>"
  Bus Selector6/1 -> Simple Longitudinal Wheel/3  "<VehSpd>"
  Bus Selector7/2 -> Simple Longitudinal Wheel1/4  "<FrcZ>"
  Two-Way Connection6/1 -> Bus Selector6/1, Bus Selector7/1
  Add2/1 -> Bus Creator5/1  "FrcX"
  Simple Longitudinal Wheel1/2 -> Add2/2  "Spd"
  Bus Creator5/1 -> Two-Way Connection6/1
  Simple Longitudinal Wheel/3 -> Bus Creator/2  "Omega3"
  Ground/1 -> Simple Longitudinal Wheel1/2, Simple Longitudinal Wheel/2
  Simple Longitudinal Wheel1/3 -> Bus Creator/3  "Omega4"
  Simple Longitudinal Wheel1/1 -> Terminator3/1
  connections:
  DiffAxle/RConn1 -- Two-Way Connection6/RConn1

== system EV6_LUT_FourWheel_EV6Battery77p4kWh_PowerCorrected/Vehicle Under Test1/Vehicle/Vehicle Dynamics/Vehicle Longitudinal/Vehicle Body/Logitudinal Vehicle Body ==
  RoadGrade : Inport
  WindVel : Inport  Port=2  Unit=m/s
  Bus Creator : BusCreator  Inputs=2
  Bus Creator1 : BusCreator  Inputs=2
  Bus Selector : BusSelector  OutputSignals=FrcX
  Bus Selector1 : BusSelector  OutputSignals=BdyFrm.Cg.Vel.xdot,BdyFrm.Cg.Disp.x
  Bus Selector3 : BusSelector  OutputSignals=FrcX
  Signal Specification3 : SignalSpecification  Unit=N
  Signal Specification4 : SignalSpecification  Unit=N
  Transfer Fcn : TransferFcn  Denominator=[0.01 1]
  Transfer Fcn1 : TransferFcn  Denominator=[0.01 1]
  Two-Way Connection2 : TwoWayConnection
  Two-Way Connection8 : TwoWayConnection
  Unit Conversion : UnitConversion
  Vehicle Body 1DOF Longitudinal : autolibshared/Vehicle Body 1DOF Longitudinal  VariantControl=SL  extFMode=off  extMMode=off  extTamb=off  wind3D=off  aMode=1  NF=ChassisNumFrontWhls  NR=ChassisNumRearWhls  m=ChassisVehMass  a=ChassisDistCg2FrontAxle  b=ChassisDistCg2RearAxle  h=ChassisCgHeight  Cd=ChassisDragCoeff  Cl=0  Cpm=0  Af=ChassisFrontalArea  x_o=0  xdot_o=InitStates(TestScnrioCycleNum).VehSpd  Pabs=EnvPrs  T=EnvTemp  g=EnvGravCnst
      settings: LibrarySourceBlock=autolibvehdynlong/Vehicle Body 1DOF Longitudinal
  Front : PMIOPort  Side=Left
  Rear : PMIOPort  Port=2  Side=Left
  VehSpd : Outport  VectorParamsAs1DForOutWhenUnconnected=off
  VehDist : Outport  Port=2  VectorParamsAs1DForOutWhenUnconnected=off
  FrontAxleFrc : Outport  Port=3  VectorParamsAs1DForOutWhenUnconnected=off
  RearAxleFrc : Outport  Port=4  VectorParamsAs1DForOutWhenUnconnected=off
  wires:
  Bus Selector3/1 -> Transfer Fcn/1  "<FrcX>"
  Bus Creator1/1 -> Two-Way Connection2/1
  Transfer Fcn1/1 -> Signal Specification4/1
  Transfer Fcn/1 -> Signal Specification3/1
  Signal Specification4/1 -> Vehicle Body 1DOF Longitudinal/1, FrontAxleFrc/1  "FrontAxleFrc"
  Unit Conversion/1 -> Vehicle Body 1DOF Longitudinal/3
  Bus Selector1/2 -> VehDist/1  "<x>"
  Bus Selector1/1 -> VehSpd/1  "<xdot>"
  Vehicle Body 1DOF Longitudinal/4 -> Bus Creator1/2  "FrcZ"
  Two-Way Connection2/1 -> Bus Selector3/1
  WindVel/1 -> Vehicle Body 1DOF Longitudinal/4
  Vehicle Body 1DOF Longitudinal/3 -> Bus Creator/2  "FrcZ"
  Bus Creator/1 -> Two-Way Connection8/1
  Signal Specification3/1 -> Vehicle Body 1DOF Longitudinal/2, RearAxleFrc/1  "RearAxleFrc"
  Vehicle Body 1DOF Longitudinal/1 -> Bus Selector1/1  "Veh"
  Vehicle Body 1DOF Longitudinal/2 -> Bus Creator1/1, Bus Creator/1  "VehSpd"
  Bus Selector/1 -> Transfer Fcn1/1  "<FrcX>"
  RoadGrade/1 -> Unit Conversion/1
  Two-Way Connection8/1 -> Bus Selector/1
  connections:
  Two-Way Connection2/RConn1 -- Rear/RConn1
  Two-Way Connection8/RConn1 -- Front/RConn1

== system EV6_LUT_FourWheel_EV6Battery77p4kWh_PowerCorrected/Vehicle Under Test1/Vehicle/Vehicle Dynamics/Vehicle Longitudinal/Vehicle Body/Subsystem1 ==
  VehSpd : Inport
  VehDist : Inport  Port=2
  FrontAxleFrc : Inport  Port=3
  RearAxleFrc : Inport  Port=4
  Bus Creator : BusCreator  Inputs=4
  ChassisPlant : Outport
  wires:
  RearAxleFrc/1 -> Bus Creator/4  "RearAxleFrc"
  FrontAxleFrc/1 -> Bus Creator/3  "FrontAxleFrc"
  Bus Creator/1 -> ChassisPlant/1  "ChassisPlant"
  VehDist/1 -> Bus Creator/2  "VehDist"
  VehSpd/1 -> Bus Creator/1  "VehSpd"

== system EV6_LUT_FourWheel_EV6Battery77p4kWh_PowerCorrected/Vehicle Under Test1/Vehicle/Actuation and Outputs/MOOG Brake Actuator/ CAN Settings/ CAN diagnostic Counter/Timer ==
  Reset : Inport
  Constant : Constant
  Integrator : Integrator  ExternalReset=level  LimitOutput=on  LowerSaturationLimit=0  ZeroCross=off
  Timer : Outport
  wires:
  Constant/1 -> Integrator/1
  Reset/1 -> Integrator/2
  Integrator/1 -> Timer/1

== system EV6_LUT_FourWheel_EV6Battery77p4kWh_PowerCorrected/Vehicle Under Test1/Vehicle/Battery/Battery/Lithium Ion Battery Pack1/Datasheet Battery Internal/Datasheet Battery ==
  CapInit : Inport  Unit=A*hr
  BattCurr : Inport  Port=2  Unit=A
  BattTemp : Inport  Port=3  Unit=K
  Charge Model : Subsystem
  State of Charge Capacity : Subsystem
  Voltage and Power Calculation : Subsystem
  LdCurrFeed : Outport  Unit=A  VectorParamsAs1DForOutWhenUnconnected=off
  OutVoltUnfilt : Outport  Port=2  Unit=V  VectorParamsAs1DForOutWhenUnconnected=off
  LdAmpHr : Outport  Port=3  Unit=A*hr  VectorParamsAs1DForOutWhenUnconnected=off
  BattSoc : Outport  Port=4  Unit=1  VectorParamsAs1DForOutWhenUnconnected=off
  BattPwrLoss : Outport  Port=5  Unit=V  VectorParamsAs1DForOutWhenUnconnected=off
  wires:
  BattCurr/1 -> LdCurrFeed/1, Voltage and Power Calculation/2(LdAmp), Charge Model/1(LdAmp)
  Voltage and Power Calculation/1(OutVolt) -> OutVoltUnfilt/1
  Charge Model/1(LdAmpHr) -> State of Charge Capacity/1(LdAmpHr), LdAmpHr/1
  State of Charge Capacity/1(CapSOC) -> Voltage and Power Calculation/1(CapSOC), BattSoc/1
  BattTemp/1 -> Voltage and Power Calculation/3(BattTemp)
  CapInit/1 -> Charge Model/2(CapInit)
  Voltage and Power Calculation/2(BattPwrLoss) -> BattPwrLoss/1
